simulink model "kapitsa_pendulum"  (R2023b)
settings: Solver=VariableStepAuto  StartTime=0.0  StopTime=5.0  MaxStep=0.005  RelTol=1e-3
undefined symbols (not defined in the file or in its folder): I
libraries: simulink_extras x2
settings Model: Creator=LaL  LastModifiedBy=LaL

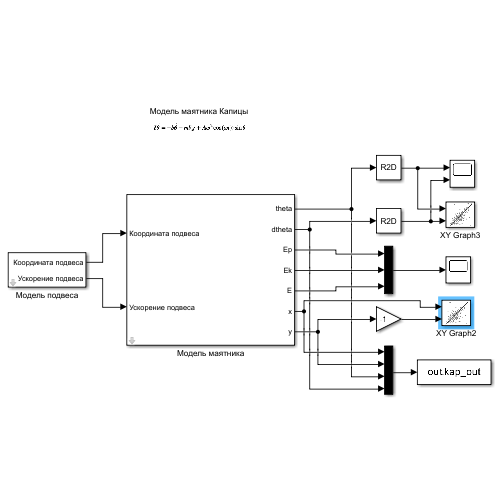
[thumbnail: Simulink's stored preview of the top-level diagram]
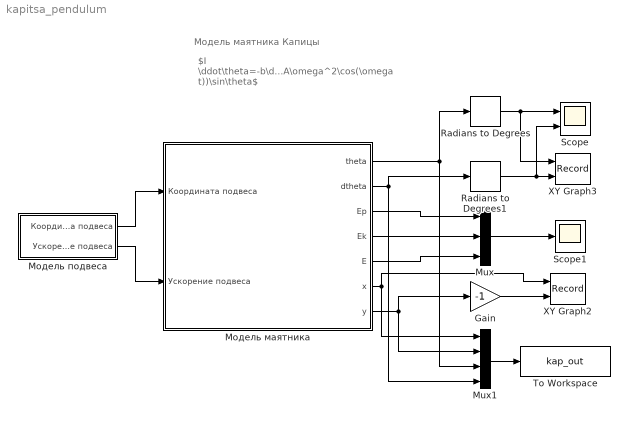
== system kapitsa_pendulum ==
  note: $I \ddot\theta=-b\dot\theta-ml(g+A\omega^2\cos(\omega t))\sin\theta$
  note: Модель маятника Капицы
  Gain : Gain  Gain=-1
  Mux : Mux  Inputs=3
  Mux1 : Mux
  Radians to Degrees : simulink_extras/Transformations/Radians to Degrees
  Radians to Degrees1 : simulink_extras/Transformations/Radians to Degrees
  Scope : Scope  NumInputPorts=2
  Scope1 : Scope
  To Workspace : ToWorkspace  VariableName=kap_out  SampleTime=-1
  XY Graph2 : Record  FileSettingsInternal="{\"entries\":[{\"content\":{\"excelSettings\":{\"content\":{},\"type\":\"Streamout.ExcelSettings\"}},\"type\":\"Streamout.FileSettingStorage\",\"uuid\":\"\"}],\"packageUris\":[\"http:\\/\\/schema.mathworks.com\\/mf0\\/streamout_blocks\\/R2020a\"],\"version\":\"1.0\"}"  Layout=[1 1]  SignalsInternal="{\"entries\":[{\"content\":{\"signals\":[{\"content\":{\"blockPath\":[],\"dimensions\":[1],\"domain\":\"\",\"lineColor\":\"#a2142f\",\"plots\":[1],\"port\":1,\"sid\":[\"\"],\"signalID\":634,\"signalName\":\"Модель маятника:6\"},\"type\":\"RecordBlkView.Signal\",\"uuid\":\"\"},{\"content\":{\"blockPath\":[],\"dimensions\":[1],\"domain\":\"\",\"lineColor\":\"#139fff\",\"plots\":[1],\"port\":2,\"sid\":[\"\"],\"signalID\":638,\"signalName\":\"Gain\"},\"type\":\"RecordBlkView.Signal\",\"uuid\":\"\"}]},\"type\":\"RecordBlkView.InputSignals\",\"uuid\":\"\"}],\"packageUris\":[\"http:\\/\\/schema.mathworks.com\\/mf0\\/streamout_blocks\\/R2020a\"],\"version\":\"1.0\"}"  VisualizationBindings="{\"xyplotplugin\":{\"info\":[{\"series\":[{\"bindingParametersList\":[{\"parameter\":\"X-Axis\",\"signalID\":634,\"signalName\":\"Модель маятника:6\"},{\"parameter\":\"Y-Axis\",\"signalID\":638,\"signalName\":\"Gain\"}],\"seriesID\":24440}],\"subplotID\":1}]}}"  CompatibilityTag=XY
  XY Graph3 : Record  FileSettingsInternal="{\"entries\":[{\"content\":{\"excelSettings\":{\"content\":{},\"type\":\"Streamout.ExcelSettings\"}},\"type\":\"Streamout.FileSettingStorage\",\"uuid\":\"\"}],\"packageUris\":[\"http:\\/\\/schema.mathworks.com\\/mf0\\/streamout_blocks\\/R2020a\"],\"version\":\"1.0\"}"  Layout=[1 1]  SignalsInternal="{\"entries\":[{\"content\":{\"signals\":[{\"content\":{\"blockPath\":[],\"dimensions\":[1],\"domain\":\"\",\"lineColor\":\"#a2142f\",\"plots\":[1],\"port\":1,\"sid\":[\"\"],\"signalID\":642,\"signalName\":\"Radians\\nto Degrees\"},\"type\":\"RecordBlkView.Signal\",\"uuid\":\"\"},{\"content\":{\"blockPath\":[],\"dimensions\":[1],\"domain\":\"\",\"lineColor\":\"#139fff\",\"plots\":[1],\"port\":2,\"sid\":[\"\"],\"signalID\":646,\"signalName\":\"Radians\\nto Degrees1\"},\"type\":\"RecordBlkView.Signal\",\"uuid\":\"\"}]},\"type\":\"RecordBlkView.InputSignals\",\"uuid\":\"\"}],\"packageUris\":[\"http:\\/\\/schema.mathworks.com\\/mf0\\/streamout_blocks\\/R2020a\"],\"version\":\"1.0\"}"  VisualizationBindings="{\"xyplotplugin\":{\"info\":[{\"series\":[{\"bindingParametersList\":[{\"parameter\":\"X-Axis\",\"signalID\":642,\"signalName\":\"Radians\\nto Degrees\"},{\"parameter\":\"Y-Axis\",\"signalID\":646,\"signalName\":\"Radians\\nto Degrees1\"}],\"seriesID\":27656}],\"subplotID\":1}]}}"  CompatibilityTag=XY
  Модель маятника : Subsystem  mask{g=9.815, m=1, l=1, b=0.3, startDegree=2.5}
      mask prompts: g "Гравитация(м/с^2)"; m "Масса груза(кг)"; l "Длина маятника(м)"; b "Декримент затухания"; startDegree "Начальный угол отклонения маятника(рад)"
  Модель подвеса : Subsystem  mask{Ap=0.1, vp=5}
      mask prompts: Ap "Амплитуда подвеса(м)"; vp "Частота подвеса(Гц)"
  wires:
  Модель маятника/5(E) -> Mux/3
  Radians to Degrees/1 -> Scope/1, XY Graph3/1
  Mux/1 -> Scope1/1
  Модель маятника/4(Ek) -> Mux/2
  Модель маятника/3(Ep) -> Mux/1
  Radians to Degrees1/1 -> XY Graph3/2, Scope/2
  Gain/1 -> XY Graph2/2
  Модель подвеса/1(Координата подвеса) -> Модель маятника/1(Координата подвеса)
  Модель подвеса/2(Ускорение подвеса) -> Модель маятника/2(Ускорение подвеса)
  Модель маятника/6(x) -> Mux1/1, XY Graph2/1
  Модель маятника/7(y) -> Mux1/2, Gain/1
  Модель маятника/2(dtheta) -> Mux1/4, Radians to Degrees1/1
  Модель маятника/1(theta) -> Mux1/3, Radians to Degrees/1
  Mux1/1 -> To Workspace/1

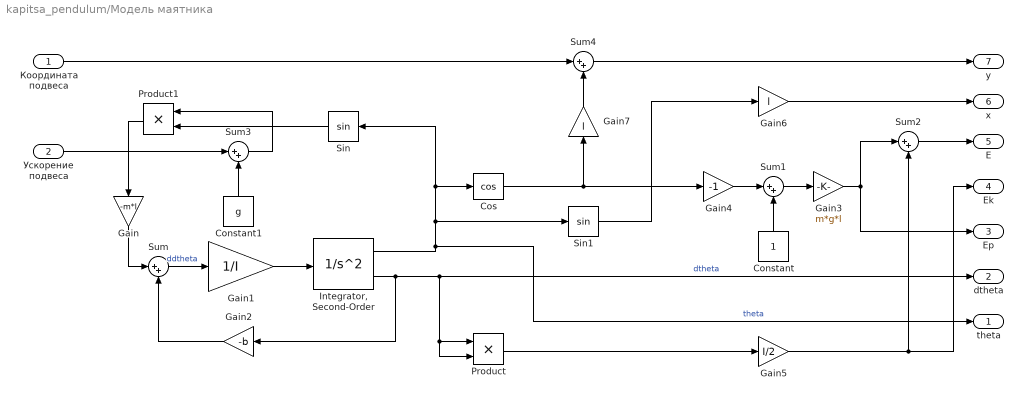
== system kapitsa_pendulum/Модель маятника ==
  Координата подвеса : Inport
  Ускорение подвеса : Inport  Port=2
  Constant : Constant
  Constant1 : Constant  Value=g
  Cos : Trigonometry  Operator=cos
  Gain : Gain  Gain=-m*l
  Gain1 : Gain  Gain=1/I
  Gain2 : Gain  Gain=-b
  Gain3 : Gain  Gain=m*g*l
  Gain4 : Gain  Gain=-1
  Gain5 : Gain  Gain=I/2
  Gain6 : Gain  Gain=l
  Gain7 : Gain  Gain=l
  "Integrator, Second-Order" : SecondOrderIntegrator  ICX=startDegree
  Product : Product
  Product1 : Product
  Sin : Trigonometry
  Sin1 : Trigonometry
  Sum{,1..4} (5 alike) : Sum  Inputs=|++
  theta : Outport
  dtheta : Outport  Port=2
  Ep : Outport  Port=3
  Ek : Outport  Port=4
  E : Outport  Port=5
  x : Outport  Port=6
  y : Outport  Port=7
  wires:
  Sin/1 -> Product1/2
  Gain/1 -> Sum/1
  "Integrator, Second-Order"/1 -> Sin/1, Cos/1, Sin1/1, theta/1  "theta"
  Gain1/1 -> "Integrator, Second-Order"/1
  "Integrator, Second-Order"/2 -> Gain2/1, Product/2, Product/1, dtheta/1  "dtheta"
  Sum/1 -> Gain1/1  "ddtheta"
  Gain2/1 -> Sum/2
  Cos/1 -> Gain4/1, Gain7/1
  Gain4/1 -> Sum1/1
  Constant/1 -> Sum1/2
  Sum1/1 -> Gain3/1
  Gain3/1 -> Ep/1, Sum2/1
  Product/1 -> Gain5/1
  Gain5/1 -> Sum2/2, Ek/1
  Sum2/1 -> E/1
  Sin1/1 -> Gain6/1
  Gain6/1 -> x/1
  Gain7/1 -> Sum4/2
  Product1/1 -> Gain/1
  Constant1/1 -> Sum3/2
  Ускорение подвеса/1 -> Sum3/1
  Sum3/1 -> Product1/1
  Sum4/1 -> y/1
  Координата подвеса/1 -> Sum4/1

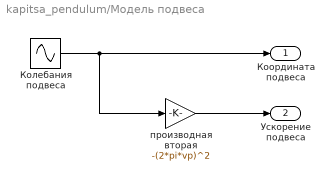
== system kapitsa_pendulum/Модель подвеса ==
  Колебания подвеса : Sin  Amplitude=Ap  Frequency=vp  Phase=pi/2  SampleTime=0
  производная вторая : Gain  Gain=-(2*pi*vp)^2
  Координата подвеса : Outport
  Ускорение подвеса : Outport  Port=2
  wires:
  Колебания подвеса/1 -> Координата подвеса/1, производная вторая/1
  производная вторая/1 -> Ускорение подвеса/1
